simulink model "Cell_3RC_Dynamic_Model"  (R2026b)
settings: Solver=ode45  StopTime=3600
values from neighbouring files (symbols this model uses):
  inv_tau1 = 1 / tau1    (= 1)    [TestModelScript.m]
  inv_tau2 = 1 / tau2    (= 0.0666666666667)    [TestModelScript.m]
  inv_tau3 = 1 / tau3    (= 0.01)    [TestModelScript.m]
  OCV_Chg_Table = [ ... (first row only)    [TestModelScript.m]
  OCV_Dis_Table = [ ... (first row only)    [TestModelScript.m]
  R0_Chg_Table = w_R0 .* DCIR_Chg_Table    [TestModelScript.m]
  R0_Dis_Table = w_R0 .* DCIR_Dis_Table    [TestModelScript.m]
  R1_Chg_Table = w_R1 .* DCIR_Chg_Table    [TestModelScript.m]
  R1_Dis_Table = w_R1 .* DCIR_Dis_Table    [TestModelScript.m]
  R2_Chg_Table = w_R2 .* DCIR_Chg_Table    [TestModelScript.m]
  R2_Dis_Table = w_R2 .* DCIR_Dis_Table    [TestModelScript.m]
  R3_Chg_Table = w_R3 .* DCIR_Chg_Table    [TestModelScript.m]
  R3_Dis_Table = w_R3 .* DCIR_Dis_Table    [TestModelScript.m]
  SOC_bp_dcir = 0:10:100    [TestModelScript.m]
  SOC_bp_ocv = 0:5:100    [TestModelScript.m]
  SOC_gain = -100 / Q_nom_As    (= -0.00578703703704)    [TestModelScript.m]
  SOC_Inv_Chg_Tbl = zeros(length(V_bp_inv), length(Temp_bp_ocv))    [TestModelScript.m]
  SOC_Inv_Dis_Tbl = zeros(length(V_bp_inv), length(Temp_bp_ocv))    [TestModelScript.m]
  Temp_bp_dcir = [-20, -10, 0, 10, 25, 45, 60]    [TestModelScript.m]
  Temp_bp_ocv = [-20, -10, 0, 10, 25, 45, 55]    [TestModelScript.m]
  Temp_default = 25.0    (= 25)    [TestModelScript.m]
  V_bp_inv = linspace(2.90, 4.16, 64)    [TestModelScript.m]
  V_init_default = 3.2    [TestModelScript.m]
settings Model: Creator=hari.r  LastModifiedBy=hari.r

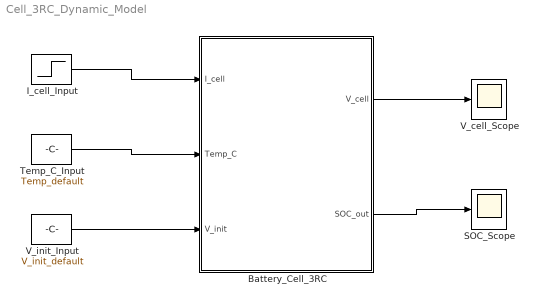
== system Cell_3RC_Dynamic_Model ==
  Battery_Cell_3RC : Subsystem
  I_cell_Input : Step  Time=10  FinalValue=4.8  SampleTime=0
  SOC_Scope : Scope
  Temp_C_Input : Constant  Value=Temp_default
  V_cell_Scope : Scope
  V_init_Input : Constant  Value=V_init_default
  wires:
  I_cell_Input/1 -> Battery_Cell_3RC/1(I_cell)
  Temp_C_Input/1 -> Battery_Cell_3RC/2(Temp_C)
  V_init_Input/1 -> Battery_Cell_3RC/3(V_init)
  Battery_Cell_3RC/1(V_cell) -> V_cell_Scope/1
  Battery_Cell_3RC/2(SOC_out) -> SOC_Scope/1

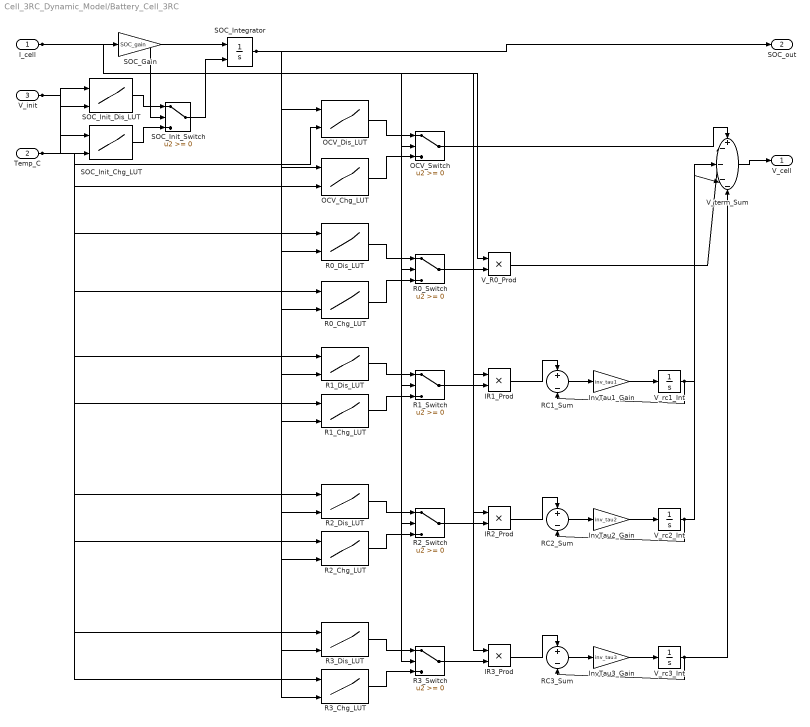
== system Cell_3RC_Dynamic_Model/Battery_Cell_3RC ==
  I_cell : Inport
  Temp_C : Inport  Port=2
  V_init : Inport  Port=3
  IR1_Prod : Product
  IR2_Prod : Product
  IR3_Prod : Product
  InvTau1_Gain : Gain  Gain=inv_tau1
  InvTau2_Gain : Gain  Gain=inv_tau2
  InvTau3_Gain : Gain  Gain=inv_tau3
  OCV_Chg_LUT : Lookup_n-D  BreakpointsForDimension1=SOC_bp_ocv  BreakpointsForDimension2=Temp_bp_ocv  Table=OCV_Chg_Table  InternalRulePriority=Speed  RndMeth=Simplest
      settings: InputPortMap=u0,u1
  OCV_Dis_LUT : Lookup_n-D  BreakpointsForDimension1=SOC_bp_ocv  BreakpointsForDimension2=Temp_bp_ocv  Table=OCV_Dis_Table  InternalRulePriority=Speed  RndMeth=Simplest
      settings: InputPortMap=u0,u1
  OCV_Switch : Switch  SaturateOnIntegerOverflow=off  InputSameDT=off
  R0_Chg_LUT : Lookup_n-D  BreakpointsForDimension1=Temp_bp_dcir  BreakpointsForDimension2=SOC_bp_dcir  Table=R0_Chg_Table  InternalRulePriority=Speed  RndMeth=Simplest
      settings: InputPortMap=u0,u1
  R0_Dis_LUT : Lookup_n-D  BreakpointsForDimension1=Temp_bp_dcir  BreakpointsForDimension2=SOC_bp_dcir  Table=R0_Dis_Table  InternalRulePriority=Speed  RndMeth=Simplest
      settings: InputPortMap=u0,u1
  R0_Switch : Switch  SaturateOnIntegerOverflow=off  InputSameDT=off
  R1_Chg_LUT : Lookup_n-D  BreakpointsForDimension1=Temp_bp_dcir  BreakpointsForDimension2=SOC_bp_dcir  Table=R1_Chg_Table  InternalRulePriority=Speed  RndMeth=Simplest
      settings: InputPortMap=u0,u1
  R1_Dis_LUT : Lookup_n-D  BreakpointsForDimension1=Temp_bp_dcir  BreakpointsForDimension2=SOC_bp_dcir  Table=R1_Dis_Table  InternalRulePriority=Speed  RndMeth=Simplest
      settings: InputPortMap=u0,u1
  R1_Switch : Switch  SaturateOnIntegerOverflow=off  InputSameDT=off
  R2_Chg_LUT : Lookup_n-D  BreakpointsForDimension1=Temp_bp_dcir  BreakpointsForDimension2=SOC_bp_dcir  Table=R2_Chg_Table  InternalRulePriority=Speed  RndMeth=Simplest
      settings: InputPortMap=u0,u1
  R2_Dis_LUT : Lookup_n-D  BreakpointsForDimension1=Temp_bp_dcir  BreakpointsForDimension2=SOC_bp_dcir  Table=R2_Dis_Table  InternalRulePriority=Speed  RndMeth=Simplest
      settings: InputPortMap=u0,u1
  R2_Switch : Switch  SaturateOnIntegerOverflow=off  InputSameDT=off
  R3_Chg_LUT : Lookup_n-D  BreakpointsForDimension1=Temp_bp_dcir  BreakpointsForDimension2=SOC_bp_dcir  Table=R3_Chg_Table  InternalRulePriority=Speed  RndMeth=Simplest
      settings: InputPortMap=u0,u1
  R3_Dis_LUT : Lookup_n-D  BreakpointsForDimension1=Temp_bp_dcir  BreakpointsForDimension2=SOC_bp_dcir  Table=R3_Dis_Table  InternalRulePriority=Speed  RndMeth=Simplest
      settings: InputPortMap=u0,u1
  R3_Switch : Switch  SaturateOnIntegerOverflow=off  InputSameDT=off
  RC1_Sum : Sum  Inputs=+-
  RC2_Sum : Sum  Inputs=+-
  RC3_Sum : Sum  Inputs=+-
  SOC_Gain : Gain  Gain=SOC_gain
  SOC_Init_Chg_LUT : Lookup_n-D  BreakpointsForDimension1=V_bp_inv  BreakpointsForDimension2=Temp_bp_ocv  Table=SOC_Inv_Chg_Tbl  InternalRulePriority=Speed  RndMeth=Simplest
      settings: InputPortMap=u0,u1
  SOC_Init_Dis_LUT : Lookup_n-D  BreakpointsForDimension1=V_bp_inv  BreakpointsForDimension2=Temp_bp_ocv  Table=SOC_Inv_Dis_Tbl  InternalRulePriority=Speed  RndMeth=Simplest
      settings: InputPortMap=u0,u1
  SOC_Init_Switch : Switch  SaturateOnIntegerOverflow=off  InputSameDT=off
  SOC_Integrator : Integrator  InitialConditionSource=external  LimitOutput=on  UpperSaturationLimit=100  LowerSaturationLimit=0
  V_R0_Prod : Product
  V_rc1_Int : Integrator
  V_rc2_Int : Integrator
  V_rc3_Int : Integrator
  V_term_Sum : Sum  Inputs=+----
  V_cell : Outport
  SOC_out : Outport  Port=2
  wires:
  V_init/1 -> SOC_Init_Dis_LUT/1, SOC_Init_Chg_LUT/1
  Temp_C/1 -> SOC_Init_Dis_LUT/2, SOC_Init_Chg_LUT/2, OCV_Dis_LUT/2, OCV_Chg_LUT/2, R0_Dis_LUT/1, R0_Chg_LUT/1, R1_Dis_LUT/1, R1_Chg_LUT/1, R2_Dis_LUT/1, R2_Chg_LUT/1, R3_Dis_LUT/1, R3_Chg_LUT/1
  SOC_Init_Dis_LUT/1 -> SOC_Init_Switch/1
  I_cell/1 -> SOC_Init_Switch/2, SOC_Gain/1, OCV_Switch/2, R0_Switch/2, V_R0_Prod/1, R1_Switch/2, IR1_Prod/1, R2_Switch/2, IR2_Prod/1, R3_Switch/2, IR3_Prod/1
  SOC_Init_Chg_LUT/1 -> SOC_Init_Switch/3
  SOC_Gain/1 -> SOC_Integrator/1
  SOC_Init_Switch/1 -> SOC_Integrator/2
  SOC_Integrator/1 -> SOC_out/1, OCV_Dis_LUT/1, OCV_Chg_LUT/1, R0_Dis_LUT/2, R0_Chg_LUT/2, R1_Dis_LUT/2, R1_Chg_LUT/2, R2_Dis_LUT/2, R2_Chg_LUT/2, R3_Dis_LUT/2, R3_Chg_LUT/2
  OCV_Dis_LUT/1 -> OCV_Switch/1
  OCV_Chg_LUT/1 -> OCV_Switch/3
  R0_Dis_LUT/1 -> R0_Switch/1
  R0_Chg_LUT/1 -> R0_Switch/3
  R0_Switch/1 -> V_R0_Prod/2
  R1_Dis_LUT/1 -> R1_Switch/1
  R1_Chg_LUT/1 -> R1_Switch/3
  R1_Switch/1 -> IR1_Prod/2
  IR1_Prod/1 -> RC1_Sum/1
  V_rc1_Int/1 -> RC1_Sum/2, V_term_Sum/3
  RC1_Sum/1 -> InvTau1_Gain/1
  InvTau1_Gain/1 -> V_rc1_Int/1
  R2_Dis_LUT/1 -> R2_Switch/1
  R2_Chg_LUT/1 -> R2_Switch/3
  R2_Switch/1 -> IR2_Prod/2
  IR2_Prod/1 -> RC2_Sum/1
  V_rc2_Int/1 -> RC2_Sum/2, V_term_Sum/4
  RC2_Sum/1 -> InvTau2_Gain/1
  InvTau2_Gain/1 -> V_rc2_Int/1
  R3_Dis_LUT/1 -> R3_Switch/1
  R3_Chg_LUT/1 -> R3_Switch/3
  R3_Switch/1 -> IR3_Prod/2
  IR3_Prod/1 -> RC3_Sum/1
  V_rc3_Int/1 -> RC3_Sum/2, V_term_Sum/5
  RC3_Sum/1 -> InvTau3_Gain/1
  InvTau3_Gain/1 -> V_rc3_Int/1
  OCV_Switch/1 -> V_term_Sum/1
  V_R0_Prod/1 -> V_term_Sum/2
  V_term_Sum/1 -> V_cell/1
